simulink model "mpc_ttype_psm"  (R2026a)
settings: Solver=ode23tb  StopTime=param.sim.simlength  FixedStep=param.glb_time.tc  MaxStep=param.glb_time.tc
values from neighbouring files (symbols this model uses):
  param = struct()    [init_model.m]
libraries: fl_lib x25, nesl_utility x12, cstblocks_lti x6, lithium_ion_battery x1, dclink_for_three_levels x1, three_phase_three_level_ttype_inverter_ideal_switch_based_model x1, single_phase_pwm_modulator x1, threephase_inductor_lib x1, simple_flexible_shaft x1, permanent_magnet_synchronous_machine x1
(part 4 of 4)

== matlab function mpc_ttype_psm/inv_psm_mod1/inverter_ctrl/inverter_control/inner_ctrl/mp control/mpc_pu_d ==
  data: S1a output; S2a output; S3a output; S4a output; S1b output; S2b output; S3b output; S4b output; S1c output; S2c output; S3c output; S4c output; vdc1 input; vdc2 input; ialpha_ref input; ibeta_ref input; ialpha input; ualpha output; ibeta input; omega_hat input; psi_alpha_hat input; psi_beta_hat input; ubeta output; L_norm input; R_norm input; u_scale input; np_gain input; k_kalman input; k_dc input; k_sw input; ts_pu input
function [S1a, S2a, S3a, S4a, S1b, S2b, S3b, S4b, S1c, S2c, S3c, S4c, ualpha, ubeta] = mpc_ttype_gate(...
    vdc1, vdc2, ialpha_ref, ibeta_ref, ialpha, ibeta, ...
    omega_hat, psi_alpha_hat, psi_beta_hat, L_norm, R_norm, u_scale, ...
    np_gain, k_kalman, k_dc, k_sw, ts_pu)
% Finite-set predictive current control of the three-level T-type bridge: every control step it tests the
% 27 states of the bridge and applies the one with the lowest cost (current error, neutral point, switching).
%
% Inputs, all per unit:
%   vdc1, vdc2              voltages of the upper and lower DC-link capacitors, pu of udc_nom
%   ialpha_ref, ibeta_ref   current reference, pu of ibez
%   ialpha, ibeta           current measured one control step before, pu of ibez
%   omega_hat               speed of the EKF, pu of omega_bez
%   psi_alpha_hat, psi_beta_hat   flux of the EKF, pu of psi_m
%   L_norm, R_norm          inductance and resistance seen by the bridge: q axis of the machine plus the output
%                           inductor, pu of the machine (the EKF uses the same values)
%   u_scale                 udc_nom/ubez: voltage in pu of udc_nom -> voltage in pu of ubez
%   np_gain                 ibez/(C*udc_nom*omega_bez), C = one capacitor of the DC link: change of vdc1 - vdc2
%                           (pu of udc_nom) for 1 pu of neutral-point current during 1 pu of time
%   k_kalman, k_dc, k_sw    weights of the current error, of vdc1 - vdc2 and of the number of level changes of
%                           the legs (switching: O<->P and O<->N count 1, P<->N counts 2)
%   ts_pu                   control step in pu of time (ts*omega_bez)
% Outputs:
%   S1a ... S4c             gate commands (0 or 15 V) of Q1 ... Q4 of the legs a, b, c:
%                           P = Q1 + Q2, O = Q2 + Q3, N = Q3 + Q4 (the dead time is added in the inverter)
%   ualpha, ubeta           voltage of the vector applied two control steps before, pu of ubez. It is the vector
%                           that acted before the current measured one step before: the EKF needs this pair.
%
% Timing: current and DC voltages are measured one control step before (inputs ialpha, ibeta, vdc1, vdc2), and
% the vector chosen now acts until the next step. So the control first computes the current and vdc1 - vdc2 of
% now with the vector of the last step (delay compensation), then chooses the vector for the next step.

    persistent states_table u_last u_last2 s_last

    if isempty(states_table)
        % the 27 states [leg a, leg b, leg c]: 1 = P, 0 = O (neutral point), -1 = N
        states_table = [
            -1,-1,-1; -1,-1, 0; -1,-1, 1; -1, 0,-1; -1, 0, 0; -1, 0, 1; -1, 1,-1; -1, 1, 0; -1, 1, 1;
             0,-1,-1;  0,-1, 0;  0,-1, 1;  0, 0,-1;  0, 0, 0;  0, 0, 1;  0, 1,-1;  0, 1, 0;  0, 1, 1;
             1,-1,-1;  1,-1, 0;  1,-1, 1;  1, 0,-1;  1, 0, 0;  1, 0, 1;  1, 1,-1;  1, 1, 0;  1, 1, 1
        ];
        u_last = [0; 0];            % voltage of the vector applied in the last step, pu of ubez
        u_last2 = [0; 0];           % voltage of the vector applied two steps before, pu of ubez
        s_last = [0, 0, 0];         % levels of the vector applied in the last step
    end

    Vdd = 15;
    sqrt3_2 = 0.866025403784439;
    inv_sqrt3 = 0.577350269189626;
    g = ts_pu/L_norm;

    % back-EMF of the EKF flux, e = d(psi)/dt = j*omega*psi (pu of ubez)
    ealpha = -omega_hat*psi_beta_hat;
    ebeta = omega_hat*psi_alpha_hat;

    % 1. Delay compensation: current and vdc1 - vdc2 of now, from the values measured one step before and the
    %    vector applied since then. The current of the legs at O flows out of the neutral point and moves
    %    vdc1 - vdc2: d(vdc1 - vdc2)/dt = i_np/C.
    ia_m = ialpha;
    ib_m = -0.5*ialpha + sqrt3_2*ibeta;
    ic_m = -0.5*ialpha - sqrt3_2*ibeta;
    inp_last = double(s_last(1) == 0)*ia_m + double(s_last(2) == 0)*ib_m + double(s_last(3) == 0)*ic_m;
    ialpha0 = ialpha + g*(u_last(1) - R_norm*ialpha - ealpha);
    ibeta0 = ibeta + g*(u_last(2) - R_norm*ibeta - ebeta);
    dv0 = (vdc1 - vdc2) + np_gain*inp_last*ts_pu;

    % phase currents of now: they flow through the legs during the next step
    ia0 = ialpha0;
    ib0 = -0.5*ialpha0 + sqrt3_2*ibeta0;
    ic0 = -0.5*ialpha0 - sqrt3_2*ibeta0;

    % 2. Prediction and cost of the 27 states (the first state with the lowest cost wins)
    minJ = 1e18;
    best_idx = 14;
    ua_best = 0.0;
    ub_best = 0.0;

    for n = 1:27
        sa = states_table(n,1);
        sb = states_table(n,2);
        sc = states_table(n,3);

        % leg voltages to the neutral point, pu of udc_nom: vdc1 at P, 0 at O, -vdc2 at N
        va = double(sa == 1)*vdc1 - double(sa == -1)*vdc2;
        vb = double(sb == 1)*vdc1 - double(sb == -1)*vdc2;
        vc = double(sc == 1)*vdc1 - double(sc == -1)*vdc2;

        % alpha/beta voltage of the state, pu of ubez
        ua = u_scale*(va - 0.5*vb - 0.5*vc)*2/3;
        ub = u_scale*(vb - vc)*inv_sqrt3;

        % current at the next step
        ia_p = ialpha0 + g*(ua - R_norm*ialpha0 - ealpha);
        ib_p = ibeta0 + g*(ub - R_norm*ibeta0 - ebeta);

        % vdc1 - vdc2 at the next step
        inp = double(sa == 0)*ia0 + double(sb == 0)*ib0 + double(sc == 0)*ic0;
        dv = dv0 + np_gain*inp*ts_pu;

        % level changes of the legs from the vector of the last step
        nsw = abs(sa - s_last(1)) + abs(sb - s_last(2)) + abs(sc - s_last(3));

        % cost
        J = k_kalman*((ialpha_ref - ia_p)^2 + (ibeta_ref - ib_p)^2) + k_dc*dv^2 + k_sw*nsw;

        if J < minJ
            minJ = J;
            best_idx = n;
            ua_best = ua;
            ub_best = ub;
        end
    end

    % 3. Voltage for the EKF (vector applied two steps before), then the memory of the applied vectors
    ualpha = u_last2(1);
    ubeta = u_last2(2);
    u_last2 = u_last;
    u_last = [ua_best; ub_best];
    s_last = states_table(best_idx, :);

    % 4. Gate commands of the chosen state
    ga = states_table(best_idx, 1);
    gb = states_table(best_idx, 2);
    gc = states_table(best_idx, 3);

    S1a = Vdd*double(ga == 1); S2a = Vdd*double(ga >= 0); S3a = Vdd*double(ga <= 0); S4a = Vdd*double(ga == -1);
    S1b = Vdd*double(gb == 1); S2b = Vdd*double(gb >= 0); S3b = Vdd*double(gb <= 0); S4b = Vdd*double(gb == -1);
    S1c = Vdd*double(gc == 1); S2c = Vdd*double(gc >= 0); S3c = Vdd*double(gc <= 0); S4c = Vdd*double(gc == -1);
end
